simulink model "snap_adc5g_spec_rpi"  (R2019a)
settings: Solver=VariableStepDiscrete  StartTime=0.0  StopTime=10.0  RelTol=1e-3
undefined symbols (not defined in the file): pfb_coeff_gen_calc
libraries: xbsIndex_r4 x13965, casper_library_misc x80, casper_library_delays x43, xps_library x5, xbsReplacements_r4 x2, casper_library_communications x1
(part 25 of 152)

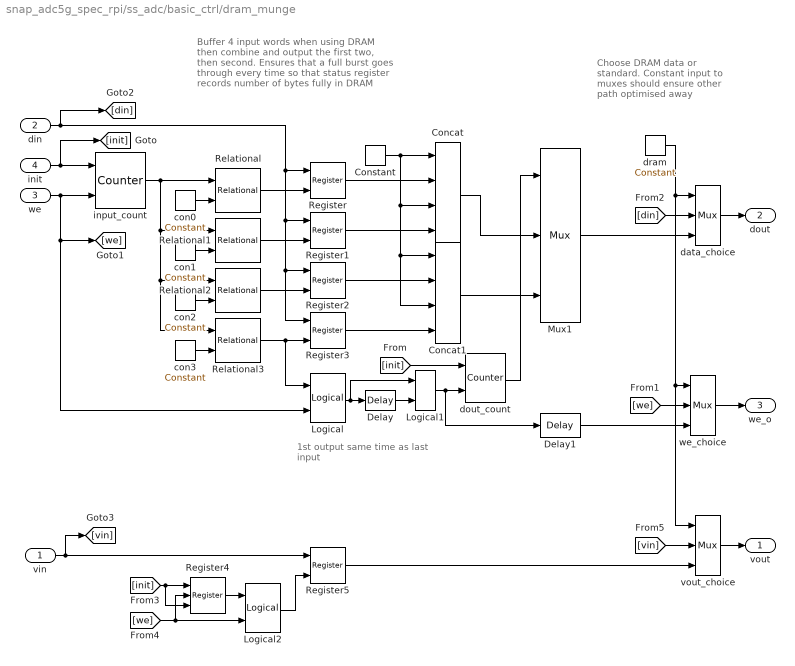
== system snap_adc5g_spec_rpi/ss_adc/basic_ctrl/dram_munge ==
  note: Buffer 4 input words when using DRAM
      | then combine and output the first two,
      | then second. Ensures that a full burst
      | goes through every time so that status
      | register records number of bytes fully in
      | DRAM
  note: Choose DRAM data
      | or standard. Constant input
      | to muxes should ensure
      | other path optimised
      | away
  note: 1st output same time
      | as last input
  vin : Inport
  din : Inport  Port=2
  we : Inport  Port=3
  init : Inport  Port=4
  Concat : xbsIndex_r4/Concat  num_inputs=4  dbl_ovrd=off  block_type=concat
  Concat1 : xbsIndex_r4/Concat  num_inputs=4  dbl_ovrd=off  block_type=concat
  Constant : xbsIndex_r4/Constant  const=0  gui_display_data_type=Fixed-point  arith_type=Unsigned  n_bits=8  bin_pt=0  preci_type=Single  exp_width=8  frac_width=24  explicit_period=on  period=1  equ=P=C  opselect=C  inp2=PCIN>>17  opr=+  inp1=P  carry=CIN  dbl_ovrd=off  block_type=constant
      settings: block_version=11.4
  Delay : xbsIndex_r4/Delay  rst=off  infoeditControl=Selection of Reset will increase slice count due to use of real FFs and instead of SRLs  en=off  latency=1  reg_retiming=off  dbl_ovrd=off  block_type=delay
      settings: block_version=11.4
  Delay1 : xbsIndex_r4/Delay  rst=off  infoeditControl=Selection of Reset will increase slice count due to use of real FFs and instead of SRLs  en=off  latency=1  reg_retiming=off  dbl_ovrd=off  block_type=delay
      settings: block_version=11.4
  Logical : xbsIndex_r4/Logical  logical_function=AND  inputs=2  en=off  latency=1  precision=Full  arith_type=Unsigned  n_bits=16  bin_pt=0  align_bp=on  dbl_ovrd=off  block_type=logical
      settings: block_version=11.4
  Logical1 : xbsIndex_r4/Logical  logical_function=OR  inputs=2  en=off  latency=0  precision=Full  arith_type=Unsigned  n_bits=16  bin_pt=0  align_bp=on  dbl_ovrd=off  block_type=logical
      settings: block_version=11.4
  Logical2 : xbsIndex_r4/Logical  logical_function=AND  inputs=2  en=off  latency=0  precision=Full  arith_type=Unsigned  n_bits=16  bin_pt=0  align_bp=on  dbl_ovrd=off  block_type=logical
      settings: block_version=11.4
  Mux1 : xbsIndex_r4/Mux  inputs=2  en=off  latency=1  precision=Full  arith_type=Unsigned  n_bits=16  bin_pt=14  quantization=Truncate  overflow=Wrap  dbl_ovrd=off  block_type=mux
      settings: block_version=11.4
  Register{,1..3,5} (5 alike) : xbsIndex_r4/Register  init=0  rst=off  en=on  dbl_ovrd=off  block_type=register
      settings: block_version=11.4
  Register4 : xbsIndex_r4/Register  init=0  rst=on  en=on  dbl_ovrd=off  block_type=register
      settings: block_version=11.4
  Relational{,1..3} (4 alike) : xbsIndex_r4/Relational  mode=a=b  op_type=Bool  en=off  latency=0  dbl_ovrd=off  block_type=relational
  con0 : xbsIndex_r4/Constant  const=0  gui_display_data_type=Fixed-point  arith_type=Unsigned  n_bits=2  bin_pt=0  preci_type=Single  exp_width=8  frac_width=24  explicit_period=on  period=1  equ=P=C  opselect=C  inp2=PCIN>>17  opr=+  inp1=P  carry=CIN  dbl_ovrd=off  block_type=constant
      settings: block_version=11.4
  con1 : xbsIndex_r4/Constant  const=1  gui_display_data_type=Fixed-point  arith_type=Unsigned  n_bits=2  bin_pt=0  preci_type=Single  exp_width=8  frac_width=24  explicit_period=on  period=1  equ=P=C  opselect=C  inp2=PCIN>>17  opr=+  inp1=P  carry=CIN  dbl_ovrd=off  block_type=constant
      settings: block_version=11.4
  con2 : xbsIndex_r4/Constant  const=2  gui_display_data_type=Fixed-point  arith_type=Unsigned  n_bits=2  bin_pt=0  preci_type=Single  exp_width=8  frac_width=24  explicit_period=on  period=1  equ=P=C  opselect=C  inp2=PCIN>>17  opr=+  inp1=P  carry=CIN  dbl_ovrd=off  block_type=constant
      settings: block_version=11.4
  con3 : xbsIndex_r4/Constant  const=3  gui_display_data_type=Fixed-point  arith_type=Unsigned  n_bits=2  bin_pt=0  preci_type=Single  exp_width=8  frac_width=24  explicit_period=on  period=1  equ=P=C  opselect=C  inp2=PCIN>>17  opr=+  inp1=P  carry=CIN  dbl_ovrd=off  block_type=constant
      settings: block_version=11.4
  data_choice : xbsIndex_r4/Mux  inputs=2  en=off  latency=0  precision=User Defined  arith_type=Unsigned  n_bits=128  bin_pt=0  quantization=Truncate  overflow=Wrap  dbl_ovrd=off  block_type=mux
      settings: block_version=11.4
  dout_count : xbsIndex_r4/Counter  cnt_type=Free Running  cnt_to=Inf  operation=Up  start_count=0  cnt_by_val=1  arith_type=Unsigned  n_bits=1  bin_pt=0  load_pin=off  rst=on  en=on  explicit_period=on  period=1  use_behavioral_HDL=off  implementation=Fabric  dbl_ovrd=off  block_type=counter
      settings: block_version=11.4
  dram : xbsIndex_r4/Constant  const=0  gui_display_data_type=Fixed-point  arith_type=Boolean  n_bits=16  bin_pt=14  preci_type=Single  exp_width=8  frac_width=24  explicit_period=on  period=1  equ=P=C  opselect=C  inp2=PCIN>>17  opr=+  inp1=P  carry=CIN  dbl_ovrd=off  block_type=constant
      settings: block_version=11.4
  input_count : xbsIndex_r4/Counter  cnt_type=Free Running  cnt_to=Inf  operation=Up  start_count=0  cnt_by_val=1  arith_type=Unsigned  n_bits=2  bin_pt=0  load_pin=off  rst=on  en=on  explicit_period=on  period=1  use_behavioral_HDL=off  implementation=Fabric  dbl_ovrd=off  block_type=counter
      settings: block_version=11.4
  vout_choice : xbsIndex_r4/Mux  inputs=2  en=off  latency=0  precision=Full  arith_type=Unsigned  n_bits=16  bin_pt=14  quantization=Truncate  overflow=Wrap  dbl_ovrd=off  block_type=mux
      settings: block_version=11.4
  we_choice : xbsIndex_r4/Mux  inputs=2  en=off  latency=0  precision=Full  arith_type=Unsigned  n_bits=16  bin_pt=14  quantization=Truncate  overflow=Wrap  dbl_ovrd=off  block_type=mux
      settings: block_version=11.4
  vout : Outport
  dout : Outport  Port=2
  we_o : Outport  Port=3
  wires:
  data_choice/1 -> dout/1
  init/1 -> input_count/1, [init]
  we/1 -> input_count/2, Logical/2, [we]
  din/1 -> Register/1, Register1/1, Register2/1, Register3/1, [din]
  input_count/1 -> Relational/1, Relational1/1, Relational2/1, Relational3/1
  con0/1 -> Relational/2
  con1/1 -> Relational1/2
  con2/1 -> Relational2/2
  con3/1 -> Relational3/2
  Relational/1 -> Register/2
  Relational1/1 -> Register1/2
  Relational2/1 -> Register2/2
  Relational3/1 -> Register3/2, Logical/1
  Logical/1 -> Delay/1, Logical1/1
  Delay/1 -> Logical1/2
  Concat/1 -> Mux1/2
  Concat1/1 -> Mux1/3
  Logical1/1 -> dout_count/2, Delay1/1
  [init] -> dout_count/1
  dout_count/1 -> Mux1/1
  we_choice/1 -> we_o/1
  Delay1/1 -> we_choice/3
  [we] -> we_choice/2
  Mux1/1 -> data_choice/3
  [din] -> data_choice/2
  dram/1 -> data_choice/1, we_choice/1, vout_choice/1
  [init] -> Register4/1, Register4/3
  Register4/1 -> Logical2/1
  vin/1 -> Register5/1, [vin]
  [we] -> Register4/2, Logical2/2
  Logical2/1 -> Register5/2
  vout_choice/1 -> vout/1
  Register5/1 -> vout_choice/3
  [vin] -> vout_choice/2
  Register/1 -> Concat/2
  Register1/1 -> Concat/4
  Constant/1 -> Concat/1, Concat/3, Concat1/1, Concat1/3
  Register2/1 -> Concat1/2
  Register3/1 -> Concat1/4

== system snap_adc5g_spec_rpi/ss_adc/bram/calc_add ==
  note: Use behavioural HDL
      | so that gets optimised
      | to minimum logic
  note: If reading/writing words
      | smaller than 32 bits,
      | change address so
      | that addressing is
      | big endian instead of
      | little, otherwise
      | pass through
  in : Inport
  add_sub : xbsIndex_r4/AddSub  mode=Subtraction  use_carryin=off  use_carryout=off  en=off  latency=0  precision=User Defined  arith_type=Unsigned  n_bits=max(1, log2(32/data_width))  bin_pt=0  quantization=Truncate  overflow=Wrap  use_behavioral_HDL=on  hw_selection=Fabric  pipelined=off  dbl_ovrd=off  block_type=addsub
  concat : xbsIndex_r4/Concat  num_inputs=2  dbl_ovrd=off  block_type=concat
  const : xbsIndex_r4/Constant  const=max(0, 32/data_width-1)  gui_display_data_type=Fixed-point  arith_type=Unsigned  n_bits=max(1, log2(32/data_width))  bin_pt=0  preci_type=Single  exp_width=8  frac_width=24  explicit_period=on  period=sample_rate  equ=P=C  opselect=C  inp2=PCIN>>17  opr=+  inp1=P  carry=CIN  dbl_ovrd=off  block_type=constant
      settings: block_version=11.4
  convert_addr : xbsIndex_r4/Convert  gui_display_data_type=Fixed-point  arith_type=Unsigned  n_bits=addr_width  bin_pt=0  float_type=Single  exp_bits=8  fraction_bits=24  quantization=Truncate  overflow=Wrap  en=off  latency=0  pipeline=off  dbl_ovrd=off  block_type=convert
      settings: xl_area=[0, 0, 0, 0, 0, 0, 0]
  lsw : xbsIndex_r4/Slice  nbits=max(1, log2(32/data_width))  boolean_output=off  mode=Lower Bit Location + Width  bit1=0  base1=MSB of Input  bit0=0  base0=LSB of Input  dbl_ovrd=off  block_type=slice
  manipulate : xbsIndex_r4/Constant  const=min(1, floor(32/data_width) - 1)  gui_display_data_type=Fixed-point  arith_type=Unsigned  n_bits=1  bin_pt=0  preci_type=Single  exp_width=8  frac_width=24  explicit_period=on  period=sample_rate  equ=P=C  opselect=C  inp2=PCIN>>17  opr=+  inp1=P  carry=CIN  dbl_ovrd=off  block_type=constant
      settings: block_version=11.4
  msw : xbsIndex_r4/Slice  nbits=addr_width - max(1, log2(32/data_width))  boolean_output=off  mode=Upper Bit Location + Width  bit1=0  base1=MSB of Input  bit0=0  base0=LSB of Input  dbl_ovrd=off  block_type=slice
  mux : xbsIndex_r4/Mux  inputs=2  en=off  latency=0  precision=Full  arith_type=Unsigned  n_bits=16  bin_pt=14  quantization=Truncate  overflow=Wrap  dbl_ovrd=off  block_type=mux
      settings: block_version=11.4
  out : Outport
  wires:
  convert_addr/1 -> mux/2, msw/1, lsw/1
  const/1 -> add_sub/1
  lsw/1 -> add_sub/2
  mux/1 -> out/1
  manipulate/1 -> mux/1
  concat/1 -> mux/3
  msw/1 -> concat/1
  add_sub/1 -> concat/2
  in/1 -> convert_addr/1

== system snap_adc5g_spec_rpi/ss_adc/bram/munge_in ==
  din : Inport
  join : Subsystem  AncestorBlock=casper_library_flow_control/bus_create  mask(bus_create){inputNum=4}
      mask prompts: inputNum "Number of inputs:"
      mask init:
      | bus_create_init(gcb,...
      |     'inputNum', inputNum);
  reinterpret : xbsIndex_r4/Reinterpret  force_arith_type=on  arith_type=Unsigned  force_bin_pt=on  bin_pt=0  block_type=reinterpret
  reinterpret_out : xbsIndex_r4/Reinterpret  force_arith_type=on  arith_type=Unsigned  force_bin_pt=on  bin_pt=0  block_type=reinterpret
  split : Subsystem  AncestorBlock=casper_library_flow_control/bus_expand  mask(bus_expand){mode=divisions of arbitrary size, outputNum=1, outputWidth=[32 32 32 32], outputBinaryPt=[0 0 0 0], outputArithmeticType=[0 0 0 0], show_format=off, outputToWorkspace=off, variablePrefix=out, outputToModelAsWell=on}
      mask prompts: outputNum "Number of outputs:"; outputWidth "Output width [msb ... lsb]:"; outputBinaryPt "Output binary point position [msb ... lsb]:"; outputArithmeticType "Output arithmetic type (ufix=0, fix=1, bool=2) [msb ... lsb]:"; show_format "Print format string?"; outputToWorkspace "Output to workspace?"; variablePrefix "Variable name prefix:"; outputToModelAsWell "Output to model as well?"
      mask help:
      | Expands a 'bus' made using a bus_create or Xilinx
      | concat block.
      | The input will be divided into the specified number
      | of outputs with the specified arithmetic types.
      | Divisions are made from most significant bit.
      mask init: same as snap_adc5g_spec_rpi/ss_adc/ctrl_split
      settings: AttributesFormatString=4 outputs
      mask TypeOptions mode: divisions of equal size | divisions of arbitrary size
      mask Callback mode: bus_expand_callback();
      mask Callback outputWidth: bus_expand_callback();
      mask Callback outputToWorkspace: bus_expand_callback();
  dout : Outport
  wires:
  reinterpret_out/1 -> dout/1
  din/1 -> reinterpret/1
  reinterpret/1 -> split/1(bus_in)
  join/1(bus_out) -> reinterpret_out/1
  split/4(lsb_out1) -> join/1(in1)
  split/3(out2) -> join/2(in2)
  split/2(out3) -> join/3(in3)
  split/1(msb_out4) -> join/4(in4)

== system snap_adc5g_spec_rpi/ss_adc/bram/munge_out ==
  din : Inport
  join : Subsystem  AncestorBlock=casper_library_flow_control/bus_create  mask(bus_create){inputNum=4}
      mask prompts: inputNum "Number of inputs:"
      mask init:
      | bus_create_init(gcb,...
      |     'inputNum', inputNum);
  reinterpret : xbsIndex_r4/Reinterpret  force_arith_type=on  arith_type=Unsigned  force_bin_pt=on  bin_pt=0  block_type=reinterpret
  reinterpret_out : xbsIndex_r4/Reinterpret  force_arith_type=on  arith_type=Unsigned  force_bin_pt=on  bin_pt=0  block_type=reinterpret
  split : Subsystem  AncestorBlock=casper_library_flow_control/bus_expand  mask(bus_expand){mode=divisions of arbitrary size, outputNum=1, outputWidth=[32 32 32 32], outputBinaryPt=[0 0 0 0], outputArithmeticType=[0 0 0 0], show_format=off, outputToWorkspace=off, variablePrefix=out, outputToModelAsWell=on}
      mask prompts: outputNum "Number of outputs:"; outputWidth "Output width [msb ... lsb]:"; outputBinaryPt "Output binary point position [msb ... lsb]:"; outputArithmeticType "Output arithmetic type (ufix=0, fix=1, bool=2) [msb ... lsb]:"; show_format "Print format string?"; outputToWorkspace "Output to workspace?"; variablePrefix "Variable name prefix:"; outputToModelAsWell "Output to model as well?"
      mask help:
      | Expands a 'bus' made using a bus_create or Xilinx
      | concat block.
      | The input will be divided into the specified number
      | of outputs with the specified arithmetic types.
      | Divisions are made from most significant bit.
      mask init: same as snap_adc5g_spec_rpi/ss_adc/ctrl_split
      settings: AttributesFormatString=4 outputs
      mask TypeOptions mode: divisions of equal size | divisions of arbitrary size
      mask Callback mode: bus_expand_callback();
      mask Callback outputWidth: bus_expand_callback();
      mask Callback outputToWorkspace: bus_expand_callback();
  dout : Outport
  wires:
  reinterpret_out/1 -> dout/1
  din/1 -> reinterpret/1
  reinterpret/1 -> split/1(bus_in)
  join/1(bus_out) -> reinterpret_out/1
  split/4(lsb_out1) -> join/1(in1)
  split/3(out2) -> join/2(in2)
  split/2(out3) -> join/3(in3)
  split/1(msb_out4) -> join/4(in4)

== system snap_adc5g_spec_rpi/ss_adc/bram/sim_mem ==
  addr : Inport
  data : Inport  Port=2
  we : Inport  Port=3
  Data Type Conversion : DataTypeConversion  OutDataTypeStr=single
  Data Type Conversion1 : DataTypeConversion  OutDataTypeStr=double
  Data Type Conversion2 : DataTypeConversion  OutDataTypeStr=boolean
  sfunc : M-S-Function  FunctionName=shared_bram_sim_sfunc  Parameters=depth_bits, latency, init_vals  mask{depth_bits=addr_width, latency=csp_latency, init_vals=init_vals}
      mask prompts: depth_bits "Depth (2^?):"; latency "Latency (>=1):"; init_vals "Initial values:"
      mask Callback latency:
      | latency = str2double(get_param(gcb, 'latency'));
      | if latency < 1
      |     errordlg('Cannot have latency less than one.');
      |     set_param(gcb, 'latency', '1');
      | end
  sim_addr : xbsIndex_r4/Gateway Out  inherit_from_input=off  hdl_port=off  rows=1  columns=1  UseAsDAC=off  DACChannel='1'  interface=None  automatic_assignment=on  address_offset=hex2dec('00')  intf_name=''  intf_description=''  timing_constraint=None  locs_specified=off  LOCs={}  io_standard={}  block_type=gatewayout
  sim_data : xbsIndex_r4/Gateway Out  inherit_from_input=off  hdl_port=off  rows=1  columns=1  UseAsDAC=off  DACChannel='1'  interface=None  automatic_assignment=on  address_offset=hex2dec('00')  intf_name=''  intf_description=''  timing_constraint=None  locs_specified=off  LOCs={}  io_standard={}  block_type=gatewayout
  sim_we : xbsIndex_r4/Gateway Out  inherit_from_input=off  hdl_port=off  rows=1  columns=1  UseAsDAC=off  DACChannel='1'  interface=None  automatic_assignment=on  address_offset=hex2dec('00')  intf_name=''  intf_description=''  timing_constraint=None  locs_specified=off  LOCs={}  io_standard={}  block_type=gatewayout
  data_out : Outport
  wires:
  sfunc/1 -> data_out/1  "output"
  Data Type Conversion2/1 -> sfunc/3  "we"
  Data Type Conversion1/1 -> sfunc/2  "data_in"
  Data Type Conversion/1 -> sfunc/1  "addr"
  sim_we/1 -> Data Type Conversion2/1
  sim_data/1 -> Data Type Conversion1/1
  sim_addr/1 -> Data Type Conversion/1
  we/1 -> sim_we/1
  data/1 -> sim_data/1
  addr/1 -> sim_addr/1

== system snap_adc5g_spec_rpi/tge/core/txctr ==
  out_reg : Inport
  assert_reg : xbsIndex_r4/Assert  assert_type=on  type_source=Explicitly  gui_display_data_type=Fixed-point  arith_type=Unsigned  n_bits=16  bin_pt=0  preci_type=Single  exp_width=8  frac_width=24  assert_rate=off  rate_source=Explicitly  period=1  output_port=on  block_type=assert
  cast_gw : xbsIndex_r4/Convert  gui_display_data_type=Fixed-point  arith_type=Unsigned  n_bits=32  bin_pt=0  float_type=Single  exp_bits=8  fraction_bits=24  quantization=Truncate  overflow=Wrap  en=off  latency=1  pipeline=off  dbl_ovrd=off  block_type=convert
  io_delay : xbsIndex_r4/Delay  rst=off  infoeditControl=Selection of Reset will increase slice count due to use of real FFs and instead of SRLs  en=off  latency=1  reg_retiming=on  dbl_ovrd=off  block_type=delay
  reint1 : xbsIndex_r4/Reinterpret  force_arith_type=on  arith_type=Unsigned  force_bin_pt=on  bin_pt=0  block_type=reinterpret
  sim_out : Terminator
  snap_adc5g_spec_rpi_tge_core_txctr_user_data_in : xbsIndex_r4/Gateway Out  inherit_from_input=off  hdl_port=on  rows=1  columns=1  UseAsDAC=off  DACChannel='1'  interface=None  automatic_assignment=on  address_offset=hex2dec('00')  intf_name=''  intf_description=''  timing_constraint=None  locs_specified=off  LOCs={}  io_standard={}  block_type=gatewayout
  wires:
  io_delay/1 -> cast_gw/1
  cast_gw/1 -> snap_adc5g_spec_rpi_tge_core_txctr_user_data_in/1
  snap_adc5g_spec_rpi_tge_core_txctr_user_data_in/1 -> sim_out/1
  out_reg/1 -> assert_reg/1
  assert_reg/1 -> reint1/1
  reint1/1 -> io_delay/1

== system snap_adc5g_spec_rpi/tge/core/txerrctr ==
  out_reg : Inport
  assert_reg : xbsIndex_r4/Assert  assert_type=on  type_source=Explicitly  gui_display_data_type=Fixed-point  arith_type=Unsigned  n_bits=16  bin_pt=0  preci_type=Single  exp_width=8  frac_width=24  assert_rate=off  rate_source=Explicitly  period=1  output_port=on  block_type=assert
  cast_gw : xbsIndex_r4/Convert  gui_display_data_type=Fixed-point  arith_type=Unsigned  n_bits=32  bin_pt=0  float_type=Single  exp_bits=8  fraction_bits=24  quantization=Truncate  overflow=Wrap  en=off  latency=1  pipeline=off  dbl_ovrd=off  block_type=convert
  io_delay : xbsIndex_r4/Delay  rst=off  infoeditControl=Selection of Reset will increase slice count due to use of real FFs and instead of SRLs  en=off  latency=1  reg_retiming=on  dbl_ovrd=off  block_type=delay
  reint1 : xbsIndex_r4/Reinterpret  force_arith_type=on  arith_type=Unsigned  force_bin_pt=on  bin_pt=0  block_type=reinterpret
  sim_out : Terminator
  snap_adc5g_spec_rpi_tge_core_txerrctr_user_data_in : xbsIndex_r4/Gateway Out  inherit_from_input=off  hdl_port=on  rows=1  columns=1  UseAsDAC=off  DACChannel='1'  interface=None  automatic_assignment=on  address_offset=hex2dec('00')  intf_name=''  intf_description=''  timing_constraint=None  locs_specified=off  LOCs={}  io_standard={}  block_type=gatewayout
  wires:
  io_delay/1 -> cast_gw/1
  cast_gw/1 -> snap_adc5g_spec_rpi_tge_core_txerrctr_user_data_in/1
  snap_adc5g_spec_rpi_tge_core_txerrctr_user_data_in/1 -> sim_out/1
  out_reg/1 -> assert_reg/1
  assert_reg/1 -> reint1/1
  reint1/1 -> io_delay/1

== system snap_adc5g_spec_rpi/tge/core/txfullctr ==
  out_reg : Inport
  assert_reg : xbsIndex_r4/Assert  assert_type=on  type_source=Explicitly  gui_display_data_type=Fixed-point  arith_type=Unsigned  n_bits=16  bin_pt=0  preci_type=Single  exp_width=8  frac_width=24  assert_rate=off  rate_source=Explicitly  period=1  output_port=on  block_type=assert
  cast_gw : xbsIndex_r4/Convert  gui_display_data_type=Fixed-point  arith_type=Unsigned  n_bits=32  bin_pt=0  float_type=Single  exp_bits=8  fraction_bits=24  quantization=Truncate  overflow=Wrap  en=off  latency=1  pipeline=off  dbl_ovrd=off  block_type=convert
  io_delay : xbsIndex_r4/Delay  rst=off  infoeditControl=Selection of Reset will increase slice count due to use of real FFs and instead of SRLs  en=off  latency=1  reg_retiming=on  dbl_ovrd=off  block_type=delay
  reint1 : xbsIndex_r4/Reinterpret  force_arith_type=on  arith_type=Unsigned  force_bin_pt=on  bin_pt=0  block_type=reinterpret
  sim_out : Terminator
  snap_adc5g_spec_rpi_tge_core_txfullctr_user_data_in : xbsIndex_r4/Gateway Out  inherit_from_input=off  hdl_port=on  rows=1  columns=1  UseAsDAC=off  DACChannel='1'  interface=None  automatic_assignment=on  address_offset=hex2dec('00')  intf_name=''  intf_description=''  timing_constraint=None  locs_specified=off  LOCs={}  io_standard={}  block_type=gatewayout
  wires:
  io_delay/1 -> cast_gw/1
  cast_gw/1 -> snap_adc5g_spec_rpi_tge_core_txfullctr_user_data_in/1
  snap_adc5g_spec_rpi_tge_core_txfullctr_user_data_in/1 -> sim_out/1
  out_reg/1 -> assert_reg/1
  assert_reg/1 -> reint1/1
  reint1/1 -> io_delay/1

== system snap_adc5g_spec_rpi/tge/core/txofctr ==
  out_reg : Inport
  assert_reg : xbsIndex_r4/Assert  assert_type=on  type_source=Explicitly  gui_display_data_type=Fixed-point  arith_type=Unsigned  n_bits=16  bin_pt=0  preci_type=Single  exp_width=8  frac_width=24  assert_rate=off  rate_source=Explicitly  period=1  output_port=on  block_type=assert
  cast_gw : xbsIndex_r4/Convert  gui_display_data_type=Fixed-point  arith_type=Unsigned  n_bits=32  bin_pt=0  float_type=Single  exp_bits=8  fraction_bits=24  quantization=Truncate  overflow=Wrap  en=off  latency=1  pipeline=off  dbl_ovrd=off  block_type=convert
  io_delay : xbsIndex_r4/Delay  rst=off  infoeditControl=Selection of Reset will increase slice count due to use of real FFs and instead of SRLs  en=off  latency=1  reg_retiming=on  dbl_ovrd=off  block_type=delay
  reint1 : xbsIndex_r4/Reinterpret  force_arith_type=on  arith_type=Unsigned  force_bin_pt=on  bin_pt=0  block_type=reinterpret
  sim_out : Terminator
  snap_adc5g_spec_rpi_tge_core_txofctr_user_data_in : xbsIndex_r4/Gateway Out  inherit_from_input=off  hdl_port=on  rows=1  columns=1  UseAsDAC=off  DACChannel='1'  interface=None  automatic_assignment=on  address_offset=hex2dec('00')  intf_name=''  intf_description=''  timing_constraint=None  locs_specified=off  LOCs={}  io_standard={}  block_type=gatewayout
  wires:
  io_delay/1 -> cast_gw/1
  cast_gw/1 -> snap_adc5g_spec_rpi_tge_core_txofctr_user_data_in/1
  snap_adc5g_spec_rpi_tge_core_txofctr_user_data_in/1 -> sim_out/1
  out_reg/1 -> assert_reg/1
  assert_reg/1 -> reint1/1
  reint1/1 -> io_delay/1

== system snap_adc5g_spec_rpi/tge/core/txs ==
  in_link_up : Inport
  in_led_tx : Inport  Port=2
  in_tx_full : Inport  Port=3
  in_tx_over : Inport  Port=4
  in_valid : Inport  Port=5
  in_eof : Inport  Port=6
  in_data : Inport  Port=7
  in_ip : Inport  Port=8
  we : Inport  Port=9
  trig : Inport  Port=10
  assert_data : xbsIndex_r4/Assert  assert_type=on  type_source=Explicitly  gui_display_data_type=Fixed-point  arith_type=Unsigned  n_bits=64  bin_pt=0  preci_type=Single  exp_width=8  frac_width=24  assert_rate=off  rate_source=Explicitly  period=1  output_port=on  block_type=assert
  assert_eof : xbsIndex_r4/Assert  assert_type=on  type_source=Explicitly  gui_display_data_type=Boolean  arith_type=Boolean  n_bits=1  bin_pt=0  preci_type=Single  exp_width=8  frac_width=24  assert_rate=off  rate_source=Explicitly  period=1  output_port=on  block_type=assert
  assert_ip : xbsIndex_r4/Assert  assert_type=on  type_source=Explicitly  gui_display_data_type=Fixed-point  arith_type=Unsigned  n_bits=32  bin_pt=0  preci_type=Single  exp_width=8  frac_width=24  assert_rate=off  rate_source=Explicitly  period=1  output_port=on  block_type=assert
  assert_led_tx : xbsIndex_r4/Assert  assert_type=on  type_source=Explicitly  gui_display_data_type=Boolean  arith_type=Boolean  n_bits=1  bin_pt=0  preci_type=Single  exp_width=8  frac_width=24  assert_rate=off  rate_source=Explicitly  period=1  output_port=on  block_type=assert
  assert_link_up : xbsIndex_r4/Assert  assert_type=on  type_source=Explicitly  gui_display_data_type=Boolean  arith_type=Boolean  n_bits=1  bin_pt=0  preci_type=Single  exp_width=8  frac_width=24  assert_rate=off  rate_source=Explicitly  period=1  output_port=on  block_type=assert
  assert_tx_full : xbsIndex_r4/Assert  assert_type=on  type_source=Explicitly  gui_display_data_type=Boolean  arith_type=Boolean  n_bits=1  bin_pt=0  preci_type=Single  exp_width=8  frac_width=24  assert_rate=off  rate_source=Explicitly  period=1  output_port=on  block_type=assert
  assert_tx_over : xbsIndex_r4/Assert  assert_type=on  type_source=Explicitly  gui_display_data_type=Boolean  arith_type=Boolean  n_bits=1  bin_pt=0  preci_type=Single  exp_width=8  frac_width=24  assert_rate=off  rate_source=Explicitly  period=1  output_port=on  block_type=assert
  assert_valid : xbsIndex_r4/Assert  assert_type=on  type_source=Explicitly  gui_display_data_type=Boolean  arith_type=Boolean  n_bits=1  bin_pt=0  preci_type=Single  exp_width=8  frac_width=24  assert_rate=off  rate_source=Explicitly  period=1  output_port=on  block_type=assert
  buscreate : Subsystem  AncestorBlock=casper_library_flow_control/bus_create  mask(bus_create){inputNum=8}
      mask prompts: inputNum "Number of inputs:"
      mask init:
      | bus_create_init(gcb,...
      |     'inputNum', inputNum);
  io_delay : Subsystem  AncestorBlock=casper_library_delays/pipeline  mask(pipeline){csp_latency=5}
      mask prompts: csp_latency "Latency"
      mask help:
      | An explicitly laid-out delay line to avoid mapping to SRL16s
      | for use in pipelining to help achieve timing closure.
      mask init:
      | pipeline_init(gcb,'latency',csp_latency);
      settings: AttributesFormatString=Latency = %<latency>
      mask Display:
      | port_label('input', 1, 'd');
      | port_label('output', 1, 'q');
      | disp(['Z^-', num2str(csp_latency)]);
  ss : Subsystem  Tag=casper:snapshot  AncestorBlock=casper_library_scopes/snapshot  mask(snapshot){storage=bram, dram_dimm=2, dram_clock=250, nsamples=11, data_width=128, offset=off, circap=off, value=off, ext_arm=off, ext_circ=off, provide_outputs=off, use_dsp48=on}
      mask prompts: storage "Storage medium"; dram_dimm "DRAM dimm"; dram_clock "DRAM clock rate"; nsamples "Number of Samples (2^?)"; data_width "Data width"; offset "Start delay support"; circap "Circular capture support"; value "Extra value capture support"; ext_arm "External arm support"; ext_circ "External circular capture support"; provide_outputs "Provide outputs"; use_dsp48 "Use DSP48s to implement counters"
      mask help:
      | Standard snap block, but with the following optional extras;
      |  1) Optionally delay the fabric trigger by a user-specified number of valids.
      |  2) Capture continuously after a trigger until a stop pulse is received. Data is captured into BRAM continuously, with old data being overwritten until a stop command is received. Then stop capturing when memory is filled. This enables you to get some data before and some data after the stop pulse. Use the 'tr_en_cnt' register to determine where you are in your vector. 'Addr' register's MSb now indicates 'busy capturing'.
      |  3) Optionally capture a value on an input port to a register at the same time as the first data sample.
      |  4) Implement counters using DSP48Es to save resources.
      mask init: same as snap_adc5g_spec_rpi/ss_adc
      settings: AttributesFormatString=|
      | 128 wide, 2048 deep
      | debugID: 79195835
      mask TypeOptions storage: bram | dram
      mask Callback storage: snapshot_callback();
      mask TypeOptions dram_dimm: 1 | 2 | 3 | 4
      mask TypeOptions dram_clock: 200 | 250 | 266 | 300 | 333
      mask TypeOptions data_width: 8 | 16 | 32 | 64 | 128
  trig_delay : Subsystem  AncestorBlock=casper_library_delays/pipeline  mask(pipeline){csp_latency=5}
      mask prompts: csp_latency "Latency"
      mask help:
      | An explicitly laid-out delay line to avoid mapping to SRL16s
      | for use in pipelining to help achieve timing closure.
      mask init:
      | pipeline_init(gcb,'latency',csp_latency);
      settings: AttributesFormatString=Latency = %<latency>
      mask Display:
      | port_label('input', 1, 'd');
      | port_label('output', 1, 'q');
      | disp(['Z^-', num2str(csp_latency)]);
  we_delay : Subsystem  AncestorBlock=casper_library_delays/pipeline  mask(pipeline){csp_latency=5}
      mask prompts: csp_latency "Latency"
      mask help:
      | An explicitly laid-out delay line to avoid mapping to SRL16s
      | for use in pipelining to help achieve timing closure.
      mask init:
      | pipeline_init(gcb,'latency',csp_latency);
      settings: AttributesFormatString=Latency = %<latency>
      mask Display:
      | port_label('input', 1, 'd');
      | port_label('output', 1, 'q');
      | disp(['Z^-', num2str(csp_latency)]);
  arm_out : Outport
  wires:
  ss/1(arm_out) -> arm_out/1
  buscreate/1(bus_out) -> io_delay/1(d)
  io_delay/1(q) -> ss/1(din)
  in_link_up/1 -> assert_link_up/1
  assert_link_up/1 -> buscreate/1(in1)
  in_led_tx/1 -> assert_led_tx/1
  assert_led_tx/1 -> buscreate/2(in2)
  in_tx_full/1 -> assert_tx_full/1
  assert_tx_full/1 -> buscreate/3(in3)
  in_tx_over/1 -> assert_tx_over/1
  assert_tx_over/1 -> buscreate/4(in4)
  in_valid/1 -> assert_valid/1
  assert_valid/1 -> buscreate/5(in5)
  in_eof/1 -> assert_eof/1
  assert_eof/1 -> buscreate/6(in6)
  in_data/1 -> assert_data/1
  assert_data/1 -> buscreate/7(in7)
  in_ip/1 -> assert_ip/1
  assert_ip/1 -> buscreate/8(in8)
  we/1 -> we_delay/1(d)
  we_delay/1(q) -> ss/2(we)
  trig/1 -> trig_delay/1(d)
  trig_delay/1(q) -> ss/3(trig)

== system snap_adc5g_spec_rpi/tge/core/txvldctr ==
  out_reg : Inport
  assert_reg : xbsIndex_r4/Assert  assert_type=on  type_source=Explicitly  gui_display_data_type=Fixed-point  arith_type=Unsigned  n_bits=16  bin_pt=0  preci_type=Single  exp_width=8  frac_width=24  assert_rate=off  rate_source=Explicitly  period=1  output_port=on  block_type=assert
  cast_gw : xbsIndex_r4/Convert  gui_display_data_type=Fixed-point  arith_type=Unsigned  n_bits=32  bin_pt=0  float_type=Single  exp_bits=8  fraction_bits=24  quantization=Truncate  overflow=Wrap  en=off  latency=1  pipeline=off  dbl_ovrd=off  block_type=convert
  io_delay : xbsIndex_r4/Delay  rst=off  infoeditControl=Selection of Reset will increase slice count due to use of real FFs and instead of SRLs  en=off  latency=1  reg_retiming=on  dbl_ovrd=off  block_type=delay
  reint1 : xbsIndex_r4/Reinterpret  force_arith_type=on  arith_type=Unsigned  force_bin_pt=on  bin_pt=0  block_type=reinterpret
  sim_out : Terminator
  snap_adc5g_spec_rpi_tge_core_txvldctr_user_data_in : xbsIndex_r4/Gateway Out  inherit_from_input=off  hdl_port=on  rows=1  columns=1  UseAsDAC=off  DACChannel='1'  interface=None  automatic_assignment=on  address_offset=hex2dec('00')  intf_name=''  intf_description=''  timing_constraint=None  locs_specified=off  LOCs={}  io_standard={}  block_type=gatewayout
  wires:
  io_delay/1 -> cast_gw/1
  cast_gw/1 -> snap_adc5g_spec_rpi_tge_core_txvldctr_user_data_in/1
  snap_adc5g_spec_rpi_tge_core_txvldctr_user_data_in/1 -> sim_out/1
  out_reg/1 -> assert_reg/1
  assert_reg/1 -> reint1/1
  reint1/1 -> io_delay/1

== system snap_adc5g_spec_rpi/timebase/timing/rst_gen ==
  arm : Inport
  pps_in : Inport  Port=2
  din : Inport  Port=3
  Constant : xbsIndex_r4/Constant  const=0  gui_display_data_type=Fixed-point  arith_type=Unsigned  n_bits=ceil(log2(reset_period+1))+1  bin_pt=0  preci_type=Single  exp_width=8  frac_width=24  explicit_period=on  period=1  equ=P=C  opselect=C  inp2=PCIN>>17  opr=+  inp1=P  carry=CIN  dbl_ovrd=off  block_type=constant
  Constant1 : xbsIndex_r4/Constant  const=reset_period+1  gui_display_data_type=Fixed-point  arith_type=Unsigned  n_bits=ceil(log2(reset_period+1))+1  bin_pt=0  preci_type=Single  exp_width=8  frac_width=24  explicit_period=on  period=1  equ=P=C  opselect=C  inp2=PCIN>>17  opr=+  inp1=P  carry=CIN  dbl_ovrd=off  block_type=constant
  Counter : xbsIndex_r4/Counter  cnt_type=Free Running  cnt_to=0  operation=Down  start_count=0  cnt_by_val=1  arith_type=Unsigned  n_bits=ceil(log2(reset_period+1))+1  bin_pt=0  load_pin=on  rst=off  en=on  explicit_period=on  period=1  use_behavioral_HDL=off  implementation=Fabric  use_rpm=off  dbl_ovrd=off  block_type=counter
  Delay3 : xbsIndex_r4/Delay  rst=off  infoeditControl=Selection of Reset will increase slice count due to use of real FFs and instead of SRLs  en=off  latency=1  reg_retiming=on  dbl_ovrd=off  block_type=delay
  Logical : xbsIndex_r4/Logical  logical_function=AND  inputs=2  en=off  latency=0  precision=Full  arith_type=Unsigned  n_bits=16  bin_pt=0  align_bp=on  dbl_ovrd=off  block_type=logical
  Logical1 : xbsIndex_r4/Logical  logical_function=OR  inputs=2  en=off  latency=0  precision=Full  arith_type=Unsigned  n_bits=16  bin_pt=0  align_bp=on  dbl_ovrd=off  block_type=logical
  Relational : xbsIndex_r4/Relational  mode=a>b  op_type=Bool  en=off  latency=0  dbl_ovrd=off  block_type=relational
      settings: block_version=10.1.3
  mrst : Outport
  dout : Outport  Port=2
  wires:
  arm/1 -> Logical1/1, Counter/1
  Counter/1 -> Relational/1
  Constant/1 -> Relational/2
  pps_in/1 -> Logical/1
  Relational/1 -> mrst/1, Logical/2
  din/1 -> Delay3/1
  Delay3/1 -> dout/1
  Constant1/1 -> Counter/2
  Logical1/1 -> Counter/3
  Logical/1 -> Logical1/2

== system snap_adc5g_spec_rpi/timebase/timing/sync_gen ==
  note: Resets to 3 to take into account latency of reset
  rst : Inport
  sync_period : Inport  Port=2
  din : Inport  Port=3
  Delay : xbsIndex_r4/Delay  rst=off  infoeditControl=Selection of Reset will increase slice count due to use of real FFs and instead of SRLs  en=off  latency=1  reg_retiming=off  dbl_ovrd=off  block_type=delay
  Logical : xbsIndex_r4/Logical  logical_function=OR  inputs=2  en=off  latency=1  precision=Full  arith_type=Unsigned  n_bits=16  bin_pt=0  align_bp=on  dbl_ovrd=off  block_type=logical
  Logical1 : xbsIndex_r4/Logical  logical_function=OR  inputs=2  en=off  latency=0  precision=Full  arith_type=Unsigned  n_bits=16  bin_pt=0  align_bp=on  dbl_ovrd=off  block_type=logical
  Relational : xbsIndex_r4/Relational  mode=a>=b  op_type=Bool  en=off  latency=1  dbl_ovrd=off  block_type=relational
      settings: block_version=10.1.3
  negedge : Subsystem  AncestorBlock=casper_library_misc/edge_detect  mask(edge_detect){edge=Falling, polarity=Active High, x_in=[0 0.08 0.08 0.16 0.16 0.24 0.24 0.32 0.32 0.4], y_in=[-1 -1  1  1  1  1  1  1  1  1], x_out=[0.6 0.68 0.68 0.76 0.76 0.84 0.84 0.92 0.92 1], y_out=[-1 -1  1  1 -1 -1 -1 -1 -1 -1]}
      mask prompts: edge "Edge Type"; polarity "Output Polarity"; x_in "Input X Positions"; y_in "Input Y Positions"; x_out "Output X Positions"; y_out "Output Y Positions"
      mask help: Output is active for one-cycle after each edge of the specified type (i.e. rising, falling or both).
      mask init: same as snap_adc5g_spec_rpi/sync/edge_detect
      settings: AttributesFormatString=|
      | falling edges
      | active high
      mask Help: Output is active for one-cycle after each edge of the specified type (i.e. rising, falling, or both).  Latency is zero.
      mask TypeOptions edge: Rising | Falling | Both
      mask TypeOptions polarity: Active High | Active Low
      mask Display:
      | plot(x_in_num,0.5+y_in_num*0.2);
      | plot(x_out_num,0.5+y_out_num*0.2);
  posedge1 : Subsystem  AncestorBlock=casper_library_misc/edge_detect  mask(edge_detect){edge=Rising, polarity=Active High, x_in=[0 0.08 0.08 0.16 0.16 0.24 0.24 0.32 0.32 0.4], y_in=[-1 -1  1  1  1  1  1  1  1  1], x_out=[0.6 0.68 0.68 0.76 0.76 0.84 0.84 0.92 0.92 1], y_out=[-1 -1  1  1 -1 -1 -1 -1 -1 -1]}
      mask prompts: edge "Edge Type"; polarity "Output Polarity"; x_in "Input X Positions"; y_in "Input Y Positions"; x_out "Output X Positions"; y_out "Output Y Positions"
      mask help: Output is active for one-cycle after each edge of the specified type (i.e. rising, falling or both).
      mask init: same as snap_adc5g_spec_rpi/sync/edge_detect
      settings: AttributesFormatString=|
      | rising edges
      | active high
      mask Help: Output is active for one-cycle after each edge of the specified type (i.e. rising, falling, or both).  Latency is zero.
      mask TypeOptions edge: Rising | Falling | Both
      mask TypeOptions polarity: Active High | Active Low
      mask Display:
      | plot(x_in_num,0.5+y_in_num*0.2);
      | plot(x_out_num,0.5+y_out_num*0.2);
  sync_count : xbsIndex_r4/Counter  cnt_type=Free Running  cnt_to=Inf  operation=Up  start_count=3  cnt_by_val=1  arith_type=Unsigned  n_bits=sync_gen_bits  bin_pt=0  load_pin=off  rst=on  en=off  explicit_period=on  period=1  use_behavioral_HDL=off  implementation=Fabric  use_rpm=on  dbl_ovrd=off  block_type=counter
  sync : Outport
  dout : Outport  Port=2
  wires:
  Delay/1 -> Logical/1
  posedge1/1(out) -> Logical/2, Logical1/2
  sync_period/1 -> Relational/2
  Logical1/1 -> sync/1
  negedge/1(out) -> Logical1/1
  Logical/1 -> sync_count/1
  Relational/1 -> posedge1/1(in)
  sync_count/1 -> Relational/1
  rst/1 -> Delay/1, negedge/1(in)
  din/1 -> dout/1

== system snap_adc5g_spec_rpi/vacc_ss/ss/add_gen ==
  note: To storage
  note: prevent one extra
      | write to address 0
  note: Do one
      | capture by
      | default
  note: Count of bytes in BRAM
      | as well as done signal
  note: A total count of
      | bytes written to
      | BRAM since trig
  note: Force MSbit of count
      | to be '1' by negating busy
      | as counter bit may be '0' or '1'
  vin : Inport
  din : Inport  Port=2
  we : Inport  Port=3
  go : Inport  Port=4
  cont : Inport  Port=5
  init : Inport  Port=6
  Concat : xbsIndex_r4/Concat  num_inputs=3  dbl_ovrd=off  block_type=concat
      settings: block_version=10.1.3
  Convert : xbsIndex_r4/Convert  gui_display_data_type=Fixed-point  arith_type=Unsigned  n_bits=32-nsamples-log2(increment)-1  bin_pt=0  float_type=Single  exp_bits=8  fraction_bits=24  quantization=Truncate  overflow=Wrap  en=off  latency=0  pipeline=off  dbl_ovrd=off  block_type=convert
      settings: block_version=10.1.3
  Delay{,3..6} (5 alike) : xbsIndex_r4/Delay  rst=off  infoeditControl=Selection of Reset will increase slice count due to use of real FFs and instead of SRLs  en=off  latency=1  reg_retiming=on  dbl_ovrd=off  block_type=delay
      settings: block_version=11.4
  Delay1 : xbsIndex_r4/Delay  rst=off  infoeditControl=Selection of Reset will increase slice count due to use of real FFs and instead of SRLs  en=off  latency=1  reg_retiming=off  dbl_ovrd=off  block_type=delay
      settings: block_version=11.4
  Delay2 : xbsIndex_r4/Delay  rst=off  infoeditControl=Selection of Reset will increase slice count due to use of real FFs and instead of SRLs  en=off  latency=1  reg_retiming=off  dbl_ovrd=off  block_type=delay
      settings: block_version=11.4
  Delay7 : xbsIndex_r4/Delay  rst=off  infoeditControl=Selection of Reset will increase slice count due to use of real FFs and instead of SRLs  en=off  latency=1  reg_retiming=off  dbl_ovrd=off  block_type=delay
      settings: block_version=11.4
  Inverter : xbsIndex_r4/Inverter  en=off  latency=1  dbl_ovrd=off  block_type=inv
      settings: block_version=11.4
  Inverter1 : xbsIndex_r4/Inverter  en=off  latency=0  dbl_ovrd=off  block_type=inv
      settings: block_version=11.4
  Logical1 : xbsIndex_r4/Logical  logical_function=AND  inputs=2  en=off  latency=1  precision=Full  arith_type=Unsigned  n_bits=8  bin_pt=2  align_bp=on  dbl_ovrd=off  block_type=logical
      settings: xl_area=[0, 0, 0, 0, 0, 0, 0]
  Logical2 : xbsIndex_r4/Logical  logical_function=AND  inputs=2  en=off  latency=1  precision=Full  arith_type=Unsigned  n_bits=8  bin_pt=2  align_bp=on  dbl_ovrd=off  block_type=logical
      settings: xl_area=[0, 0, 0, 0, 0, 0, 0]
  Logical4 : xbsIndex_r4/Logical  logical_function=OR  inputs=2  en=off  latency=0  precision=Full  arith_type=Unsigned  n_bits=8  bin_pt=2  align_bp=on  dbl_ovrd=off  block_type=logical
      settings: xl_area=[0, 0, 0, 0, 0, 0, 0]
  Logical6 : xbsIndex_r4/Logical  logical_function=AND  inputs=3  en=off  latency=0  precision=Full  arith_type=Unsigned  n_bits=8  bin_pt=2  align_bp=on  dbl_ovrd=off  block_type=logical
      settings: xl_area=[0, 0, 0, 0, 0, 0, 0]
  Register3 : xbsIndex_r4/Register  init=0  rst=on  en=on  dbl_ovrd=off  block_type=register
      settings: xl_area=[0, 0, 0, 0, 0, 0, 0]
  Register4 : xbsIndex_r4/Register  init=0  rst=off  en=on  dbl_ovrd=off  block_type=register
      settings: xl_area=[0, 0, 0, 0, 0, 0, 0]
  Register5 : xbsIndex_r4/Register  init=1  rst=on  en=on  dbl_ovrd=off  block_type=register
      settings: xl_area=[0, 0, 0, 0, 0, 0, 0]
  Shift : xbsIndex_r4/Shift  shift_dir=Left  shift_bits=32-nsamples-log2(increment)-1-1  en=off  latency=1  precision=Full  arith_type="Signed  (2's comp)"  n_bits=16  bin_pt=14  quantization=Truncate  overflow=Wrap  dbl_ovrd=off  block_type=shift
  add_gen : xbsIndex_r4/Counter  cnt_type=Free Running  cnt_to=1  operation=Up  start_count=0  cnt_by_val=increment  arith_type=Unsigned  n_bits=counter_size  bin_pt=0  load_pin=off  rst=on  en=on  explicit_period=on  period=1  use_behavioral_HDL=off  implementation=Fabric  use_rpm=on  dbl_ovrd=off  block_type=counter
      settings: xl_area=[0, 0, 0, 0, 0, 0, 0]
  edge_detect : Subsystem  AncestorBlock=casper_library_misc/edge_detect  mask(edge_detect){edge=Both, polarity=Active High, x_in=[0 0.08 0.08 0.16 0.16 0.24 0.24 0.32 0.32 0.4], y_in=[-1 -1  1  1  1  1 -1 -1 -1 -1], x_out=[0.6 0.68 0.68 0.76 0.76 0.84 0.84 0.92 0.92 1], y_out=[-1 -1  1  1 -1 -1  1  1 -1 -1]}
      mask prompts: edge "Edge Type"; polarity "Output Polarity"; x_in "Input X Positions"; y_in "Input Y Positions"; x_out "Output X Positions"; y_out "Output Y Positions"
      mask help: Output is active for one-cycle after each edge of the specified type (i.e. rising, falling or both).
      mask init: same as snap_adc5g_spec_rpi/sync/edge_detect
      settings: AttributesFormatString=|
      | both edges
      | active high
      mask Help: Output is active for one-cycle after each edge of the specified type (i.e. rising, falling, or both).  Latency is zero.
      mask TypeOptions edge: Rising | Falling | Both
      mask TypeOptions polarity: Active High | Active Low
      mask Display:
      | plot(x_in_num,0.5+y_in_num*0.2);
      | plot(x_out_num,0.5+y_out_num*0.2);
  edge_detect1 : Subsystem  AncestorBlock=casper_library_scopes/snapshot/add_gen/edge_detect  mask(edge_detect){edge=Both, polarity=Active High, x_in=[0 0.08 0.08 0.16 0.16 0.24 0.24 0.32 0.32 0.4], y_in=[-1 -1  1  1  1  1 -1 -1 -1 -1], x_out=[0.6 0.68 0.68 0.76 0.76 0.84 0.84 0.92 0.92 1], y_out=[-1 -1  1  1 -1 -1  1  1 -1 -1]}
      mask prompts: edge "Edge Type"; polarity "Output Polarity"; x_in "Input X Positions"; y_in "Input Y Positions"; x_out "Output X Positions"; y_out "Output Y Positions"
      mask help: Output is active for one-cycle after each edge of the specified type (i.e. rising, falling or both).
      mask init: same as snap_adc5g_spec_rpi/sync/edge_detect
      settings: AttributesFormatString=|
      | both edges
      | active high
      mask Help: Output is active for one-cycle after each edge of the specified type (i.e. rising, falling, or both).  Latency is zero.
      mask TypeOptions edge: Rising | Falling | Both
      mask TypeOptions polarity: Active High | Active Low
      mask Display:
      | plot(x_in_num,0.5+y_in_num*0.2);
      | plot(x_out_num,0.5+y_out_num*0.2);
  slice1 : xbsIndex_r4/Slice  nbits=nsamples+log2(increment)  boolean_output=off  mode=Lower Bit Location + Width  bit1=0  base1=LSB of Input  bit0=0  base0=LSB of Input  dbl_ovrd=off  block_type=slice
      settings: block_version=10.1.3
  slice2 : xbsIndex_r4/Slice  nbits=nsamples-burst_size  boolean_output=off  mode=Lower Bit Location + Width  bit1=0  base1=LSB of Input  bit0=log2(increment)+burst_size  base0=LSB of Input  dbl_ovrd=off  block_type=slice
      settings: block_version=10.1.3
  slice3 : xbsIndex_r4/Slice  nbits=1  boolean_output=on  mode=Lower Bit Location + Width  bit1=0  base1=MSB of Input  bit0=nsamples + log2(increment)  base0=LSB of Input  dbl_ovrd=off  block_type=slice
      settings: block_version=10.1.3
  vout : Outport
  add : Outport  Port=2
  dout : Outport  Port=3
  we_o : Outport  Port=4
  status : Outport  Port=5
  en_cnt : Outport  Port=6
  done : Outport  Port=7
  wires:
  edge_detect1/1(out) -> done/1
  Shift/1 -> Concat/1
  Delay/1 -> Register5/2
  Inverter1/1 -> Logical4/2
  cont/1 -> Delay3/1
  edge_detect/1(out) -> Inverter1/1, Register5/3
  Register4/1 -> vout/1
  Logical2/1 -> Register4/2
  Register3/1 -> Logical2/2
  vin/1 -> Delay5/1
  add_gen/1 -> slice2/1, slice1/1, Delay2/1, slice3/1
  Register5/1 -> Convert/1, Inverter/1, edge_detect1/1(in), Logical6/1
  slice3/1 -> edge_detect/1(in)
  init/1 -> Delay4/1
  Logical6/1 -> we_o/1, Logical2/1, Register3/2, add_gen/2
  Concat/1 -> status/1
  Convert/1 -> Shift/1
  slice2/1 -> add/1
  Delay2/1 -> en_cnt/1
  din/1 -> Delay6/1
  Delay1/1 -> Concat/3
  slice1/1 -> Delay1/1
  Inverter/1 -> Concat/2
  Logical4/1 -> Logical6/2
  we/1 -> Logical1/1
  go/1 -> Logical1/2
  Logical1/1 -> Logical6/3
  Delay7/1 -> Register4/1
  Delay3/1 -> Logical4/1, Register5/1
  Delay4/1 -> add_gen/1, Register3/3, Register3/1, Delay/1
  Delay5/1 -> Delay7/1
  Delay6/1 -> dout/1
